simulink model "sm_car"  (R2025a)
settings: Solver=ode23t  StartTime=0.0  StopTime=400  MaxStep=0.4  RelTol=1e-3  AbsTol=1e-3  EnableMultiTasking=on
PreLoadFcn:
  | % Due to usability issue in Repeating Sequence block
  | warning('off','Simulink:Masking:Invalid');
  | 
  | % Eliminate unnecessary warnings in inactive variants
  | % Warnings generated only if you click through inactive variant
  | warning('off','MATLAB:nonExistentField');
  | warning('off','Simulink:Parameters:BlkParamUndefined');
PostLoadFcn:
  | set_param([bdroot '/Vehicle'],'popup_trailer','Off')
  | warning('off','sm:sli:setup:compile:LocalSolverNotSupported')
  | %sm_car_config_maneuver(bdroot,'WOT Braking');
  | sm_car_config_vehicle(bdroot,'false');
  | sm_car_config_logging(bdroot);
InitFcn:
  | sm_car_config_camera;
  | Vehicle = sm_car_vehcfg_checkConfig(Vehicle);
  | sm_car_check_tire_model(bdroot);
StartFcn:
  | tic;
StopFcn:
  | Elapsed_Sim_Time = toc;
  | % disp(['Elapsed Sim Time = ' num2str(Elapsed_Sim_Time)]);
undefined symbols (not defined in the file): Axle1D, AxleIn, Camera, Control, Driver, Free, Init, Maneuver, Pedal, RaceFix, RaceSpin, Scene, ShaftL1, ShaftL2, ShaftR1, ShaftR2, Soft, Stiff, Visual, X, xy_data_car_side, Y, Z
libraries: sm_lib x1546, nesl_utility x528, fl_lib x480, SimscapeFluids_lib x61, sdl_lib x49, simulink x29, ee_lib x7, simulink_extras x6, Linkage_Systems x4, Tire_1x2x x4, AntiRollBar_Systems x2, Linkage_Decoupled x2
(part 2 of 79)

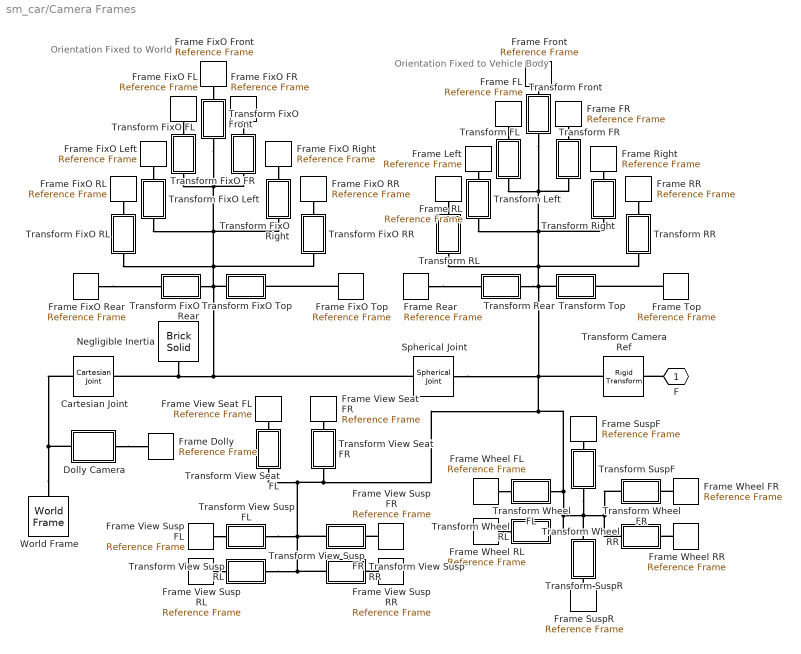
== system sm_car/Camera Frames ==
  note: Orientation Fixed to World
  note: Orientation Fixed to Vehicle Body
  Cartesian Joint : sm_lib/Joints/Cartesian Joint  JointMode=Normal  CompositeWrenchDir=FollowerOnBase  CompositeWrenchFrame=BaseFrame  SenseConstraintForce=off  SenseConstraintTorque=off  SenseTotalForce=off  SenseTotalTorque=off  PxPositionTargetSpecify=off  PxPositionTargetPriority=High  PxPositionTargetValue=0  PxPositionTargetValueUnits=m  PxVelocityTargetSpecify=off  PxVelocityTargetPriority=High  PxVelocityTargetValue=0  PxVelocityTargetValueUnits=m/s  PxEquilibriumPosition=0  PxEquilibriumPositionUnits=m  PxSpringStiffness=0  PxSpringStiffnessUnits=N/m  PxDampingCoefficient=0  PxDampingCoefficientUnits=N/(m/s)  PxLowerLimitSpecify=off  PxLowerLimitBound=-1  PxLowerLimitBoundUnits=m  PxLowerLimitStiffness=1e6  PxLowerLimitStiffnessUnits=N/m  PxLowerLimitDamping=1e3  PxLowerLimitDampingUnits=N/(m/s)  PxLowerLimitTransitionRegionWidth=1e-4  PxLowerLimitTransitionRegionWidthUnits=m  PxUpperLimitSpecify=off  PxUpperLimitBound=1  PxUpperLimitBoundUnits=m  PxUpperLimitStiffness=1e6  PxUpperLimitStiffnessUnits=N/m  PxUpperLimitDamping=1e3  PxUpperLimitDampingUnits=N/(m/s)  PxUpperLimitTransitionRegionWidth=1e-4  PxUpperLimitTransitionRegionWidthUnits=m  PxTorqueActuationMode=NoTorque  PxMotionActuationMode=ComputedMotion  PxSensePosition=off  PxSenseVelocity=off  PxSenseAcceleration=off  PxSenseTorqueForce=off  PxSenseLowerLimitTorqueForce=off  PxSenseUpperLimitTorqueForce=off  PyPositionTargetSpecify=off  PyPositionTargetPriority=High  PyPositionTargetValue=0  PyPositionTargetValueUnits=m  PyVelocityTargetSpecify=off  PyVelocityTargetPriority=High  PyVelocityTargetValue=0  PyVelocityTargetValueUnits=m/s  PyEquilibriumPosition=0  PyEquilibriumPositionUnits=m  PySpringStiffness=0  PySpringStiffnessUnits=N/m  PyDampingCoefficient=0  PyDampingCoefficientUnits=N/(m/s)  PyLowerLimitSpecify=off  PyLowerLimitBound=-1  PyLowerLimitBoundUnits=m  PyLowerLimitStiffness=1e6  PyLowerLimitStiffnessUnits=N/m  PyLowerLimitDamping=1e3  PyLowerLimitDampingUnits=N/(m/s)  PyLowerLimitTransitionRegionWidth=1e-4  PyLowerLimitTransitionRegionWidthUnits=m  PyUpperLimitSpecify=off  PyUpperLimitBound=1  PyUpperLimitBoundUnits=m  PyUpperLimitStiffness=1e6  PyUpperLimitStiffnessUnits=N/m  PyUpperLimitDamping=1e3  PyUpperLimitDampingUnits=N/(m/s)  PyUpperLimitTransitionRegionWidth=1e-4  PyUpperLimitTransitionRegionWidthUnits=m  PyTorqueActuationMode=NoTorque  PyMotionActuationMode=ComputedMotion  PySensePosition=off  PySenseVelocity=off  PySenseAcceleration=off  PySenseTorqueForce=off  PySenseLowerLimitTorqueForce=off  PySenseUpperLimitTorqueForce=off  PzPositionTargetSpecify=off  PzPositionTargetPriority=High  PzPositionTargetValue=0  PzPositionTargetValueUnits=m  PzVelocityTargetSpecify=off  PzVelocityTargetPriority=High  PzVelocityTargetValue=0  PzVelocityTargetValueUnits=m/s  PzEquilibriumPosition=0  PzEquilibriumPositionUnits=m  PzSpringStiffness=0  PzSpringStiffnessUnits=N/m  PzDampingCoefficient=0  PzDampingCoefficientUnits=N/(m/s)  PzLowerLimitSpecify=off  PzLowerLimitBound=-1  PzLowerLimitBoundUnits=m  PzLowerLimitStiffness=1e6  PzLowerLimitStiffnessUnits=N/m  PzLowerLimitDamping=1e3  PzLowerLimitDampingUnits=N/(m/s)  PzLowerLimitTransitionRegionWidth=1e-4  PzLowerLimitTransitionRegionWidthUnits=m  PzUpperLimitSpecify=off  PzUpperLimitBound=1  PzUpperLimitBoundUnits=m  PzUpperLimitStiffness=1e6  PzUpperLimitStiffnessUnits=N/m  PzUpperLimitDamping=1e3  PzUpperLimitDampingUnits=N/(m/s)  PzUpperLimitTransitionRegionWidth=1e-4  PzUpperLimitTransitionRegionWidthUnits=m  PzTorqueActuationMode=NoTorque  PzMotionActuationMode=ComputedMotion  PzSensePosition=off  PzSenseVelocity=off  PzSenseAcceleration=off  PzSenseTorqueForce=off  PzSenseLowerLimitTorqueForce=off  PzSenseUpperLimitTorqueForce=off
  Dolly Camera : Subsystem  Variant=on  VariantControlMode=label  VariantControl=Variant1  LabelModeActiveChoice=Off
      settings: AttributesFormatString=%<ActiveVariant>
      mask Display: disp(' ');
  Frame Dolly : sm_lib/Frames and Transforms/Reference Frame
  Frame FL : sm_lib/Frames and Transforms/Reference Frame
  Frame FR : sm_lib/Frames and Transforms/Reference Frame
  Frame FixO FL : sm_lib/Frames and Transforms/Reference Frame
  Frame FixO FR : sm_lib/Frames and Transforms/Reference Frame
  Frame FixO Front : sm_lib/Frames and Transforms/Reference Frame
  Frame FixO Left : sm_lib/Frames and Transforms/Reference Frame
  Frame FixO RL : sm_lib/Frames and Transforms/Reference Frame
  Frame FixO RR : sm_lib/Frames and Transforms/Reference Frame
  Frame FixO Rear : sm_lib/Frames and Transforms/Reference Frame
  Frame FixO Right : sm_lib/Frames and Transforms/Reference Frame
  Frame FixO Top : sm_lib/Frames and Transforms/Reference Frame
  Frame Front : sm_lib/Frames and Transforms/Reference Frame
  Frame Left : sm_lib/Frames and Transforms/Reference Frame
  Frame RL : sm_lib/Frames and Transforms/Reference Frame
  Frame RR : sm_lib/Frames and Transforms/Reference Frame
  Frame Rear : sm_lib/Frames and Transforms/Reference Frame
  Frame Right : sm_lib/Frames and Transforms/Reference Frame
  Frame SuspF : sm_lib/Frames and Transforms/Reference Frame
  Frame SuspR : sm_lib/Frames and Transforms/Reference Frame
  Frame Top : sm_lib/Frames and Transforms/Reference Frame
  Frame View Seat FL : sm_lib/Frames and Transforms/Reference Frame
  Frame View Seat FR : sm_lib/Frames and Transforms/Reference Frame
  Frame View Susp FL : sm_lib/Frames and Transforms/Reference Frame
  Frame View Susp FR : sm_lib/Frames and Transforms/Reference Frame
  Frame View Susp RL : sm_lib/Frames and Transforms/Reference Frame
  Frame View Susp RR : sm_lib/Frames and Transforms/Reference Frame
  Frame Wheel FL : sm_lib/Frames and Transforms/Reference Frame
  Frame Wheel FR : sm_lib/Frames and Transforms/Reference Frame
  Frame Wheel RL : sm_lib/Frames and Transforms/Reference Frame
  Frame Wheel RR : sm_lib/Frames and Transforms/Reference Frame
  Negligible Inertia : sm_lib/Body Elements/Brick Solid  BrickDimensions=[1 1 1]*1e-3  BrickDimensionsUnits=m  ExportEntireGeometry=off  InertiaType=PointMass  BasedOnType=Density  Density=1000  DensityUnits=kg/m^3  Mass=1e-6  MassUnits=kg  CenterOfMass=[0 0 0]  CenterOfMassUnits=m  MomentsOfInertia=[1 1 1]  MomentsOfInertiaUnits=kg*m^2  ProductsOfInertia=[1 1 1]  ProductsOfInertiaUnits=kg*m^2  GraphicType=FromGeometry  MarkerShape=Sphere  MarkerSize=10  GraphicVisPropType=SimpleVisualProperties  GraphicDiffuseColor=[0.5 0.5 0.5]  GraphicOpacity=1.0  GraphicSpecularColor=[0.5 0.5 0.5 1.0]  GraphicAmbientColor=[0.15 0.15 0.15 1.0]  GraphicEmissiveColor=[0.0 0.0 0.0 1.0]  GraphicShininess=75  DoExposeReferenceFrame=on  SerializedFrames=<Frames/>
  Spherical Joint : sm_lib/Joints/Spherical Joint  JointMode=Normal  CompositeWrenchDir=FollowerOnBase  CompositeWrenchFrame=BaseFrame  SenseConstraintForce=off  SenseConstraintTorque=off  SenseTotalForce=off  SenseTotalTorque=off  PositionTargetSpecify=off  PositionTargetPriority=High  PositionTargetRotationMethod=None  PositionTargetFollAlignAxisA=+X  PositionTargetBaseAlignAxisA=+Y  PositionTargetFollAlignAxisB=+Y  PositionTargetBaseAlignAxisB=+Z  PositionTargetRotationStandardAxis=+Z  PositionTargetRotationAngle=0.0  PositionTargetRotationAngleUnits=deg  PositionTargetRotationArbitraryAxis=[0 0 1]  PositionTargetRotationSequenceAxes=FollowerAxes  PositionTargetRotationSequence=XYX  PositionTargetRotationSequenceAngles=[0 0 0]  PositionTargetRotationSequenceAnglesUnits=deg  PositionTargetRotationMatrix=[1 0 0; 0 1 0; 0 0 1]  PositionTargetQuaternion=[1 0 0 0]  VelocityTargetSpecify=off  VelocityTargetPriority=High  VelocityTargetValue=[0 0 0]  VelocityTargetValueUnits=deg/s  VelocityTargetInFollowerFrame=on  EqPosRotationMethod=None  EqPosFollAlignAxisA=+X  EqPosBaseAlignAxisA=+Y  EqPosFollAlignAxisB=+Y  EqPosBaseAlignAxisB=+Z  EqPosRotationStandardAxis=+Z  EqPosRotationAngle=0.0  EqPosRotationAngleUnits=deg  EqPosRotationArbitraryAxis=[0 0 1]  EqPosRotationSequenceAxes=FollowerAxes  EqPosRotationSequence=XYX  EqPosRotationSequenceAngles=[0 0 0]  EqPosRotationSequenceAnglesUnits=deg  EqPosRotationMatrix=[1 0 0; 0 1 0; 0 0 1]  EqPosQuaternion=[1 0 0 0]  SpringStiffness=0  SpringStiffnessUnits=N*m/deg  DampingCoefficient=0  DampingCoefficientUnits=N*m/(deg/s)  LowerLimitSpecify=off  LowerLimitBound=15  LowerLimitBoundUnits=deg  LowerLimitStiffness=1e4  LowerLimitStiffnessUnits=N*m/deg  LowerLimitDamping=10  LowerLimitDampingUnits=N*m/(deg/s)  LowerLimitTransitionRegionWidth=0.1  LowerLimitTransitionRegionWidthUnits=deg  UpperLimitSpecify=off  UpperLimitBound=45  UpperLimitBoundUnits=deg  UpperLimitStiffness=1e4  UpperLimitStiffnessUnits=N*m/deg  UpperLimitDamping=10  UpperLimitDampingUnits=N*m/(deg/s)  UpperLimitTransitionRegionWidth=0.1  UpperLimitTransitionRegionWidthUnits=deg  TorqueActuationMode=NoTorque  ActuateTorqueX=off  ActuateTorqueY=off  ActuateTorqueZ=off  ActuateTorque=off  ActuationFrame=BaseFrame  SensePosition=off  SenseVelocityX=off  SenseVelocityY=off  SenseVelocityZ=off  SenseVelocity=off  SenseAccelerationX=off  SenseAccelerationY=off  SenseAccelerationZ=off  SenseAcceleration=off  SenseLowerLimitTorqueMag=off  SenseUpperLimitTorqueMag=off  SensingFrame=BaseFrame
  Transform Camera Ref : sm_lib/Frames and Transforms/Rigid Transform  RotationMethod=RotationSequence  FollAlignAxisA=+X  BaseAlignAxisA=+Y  FollAlignAxisB=+Y  BaseAlignAxisB=+Z  RotationStandardAxis=+Z  RotationAngle=0.0  RotationAngleUnits=deg  RotationArbitraryAxis=[0 0 1]  RotationSequenceAxes=FollowerAxes  RotationSequence=ZYX  RotationSequenceAngles=[Camera.Offset.a.Value(3) Camera.Offset.a.Value(2) Camera.Offset.a.Value(1)]  RotationSequenceAnglesUnits=deg  RotationMatrix=[1 0 0; 0 1 0; 0 0 1]  Quaternion=[1 0 0 0]  TranslationMethod=Cartesian  TranslationCartesianOffset=Camera.Offset.s.Value  TranslationCartesianOffsetUnits=m  TranslationStandardAxis=+Z  TranslationStandardOffset=0  TranslationStandardOffsetUnits=m  TranslationROffset=0  TranslationROffsetUnits=m  TranslationThetaOffset=0  TranslationThetaOffsetUnits=deg  TranslationZOffset=0  TranslationZOffsetUnits=m
  Transform FL : Subsystem  mask(Define Camera Frame){CF=Camera.FL}
      mask prompts: CF "Camera Frame Data (structure)"
      mask help: Sets frame position and orientation for camera frame. Data structure provides cartesian location and orientation. Orientation is intrinsic rotation of yaw-pitch-roll.
  Transform FR : Subsystem  mask(Define Camera Frame){CF=Camera.FR}
      mask prompts: CF "Camera Frame Data (structure)"
      mask help: Sets frame position and orientation for camera frame. Data structure provides cartesian location and orientation. Orientation is intrinsic rotation of yaw-pitch-roll.
  Transform FixO FL : Subsystem  mask(Define Camera Frame){CF=Camera.FL}
      mask prompts: CF "Camera Frame Data (structure)"
      mask help: Sets frame position and orientation for camera frame. Data structure provides cartesian location and orientation. Orientation is intrinsic rotation of yaw-pitch-roll.
  Transform FixO FR : Subsystem  mask(Define Camera Frame){CF=Camera.FR}
      mask prompts: CF "Camera Frame Data (structure)"
      mask help: Sets frame position and orientation for camera frame. Data structure provides cartesian location and orientation. Orientation is intrinsic rotation of yaw-pitch-roll.
  Transform FixO Front : Subsystem  mask(Define Camera Frame){CF=Camera.Front}
      mask prompts: CF "Camera Frame Data (structure)"
      mask help: Sets frame position and orientation for camera frame. Data structure provides cartesian location and orientation. Orientation is intrinsic rotation of yaw-pitch-roll.
  Transform FixO Left : Subsystem  mask(Define Camera Frame){CF=Camera.Left}
      mask prompts: CF "Camera Frame Data (structure)"
      mask help: Sets frame position and orientation for camera frame. Data structure provides cartesian location and orientation. Orientation is intrinsic rotation of yaw-pitch-roll.
  Transform FixO RL : Subsystem  mask(Define Camera Frame){CF=Camera.RL}
      mask prompts: CF "Camera Frame Data (structure)"
      mask help: Sets frame position and orientation for camera frame. Data structure provides cartesian location and orientation. Orientation is intrinsic rotation of yaw-pitch-roll.
  Transform FixO RR : Subsystem  mask(Define Camera Frame){CF=Camera.RR}
      mask prompts: CF "Camera Frame Data (structure)"
      mask help: Sets frame position and orientation for camera frame. Data structure provides cartesian location and orientation. Orientation is intrinsic rotation of yaw-pitch-roll.
  Transform FixO Rear : Subsystem  mask(Define Camera Frame){CF=Camera.Rear}
      mask prompts: CF "Camera Frame Data (structure)"
      mask help: Sets frame position and orientation for camera frame. Data structure provides cartesian location and orientation. Orientation is intrinsic rotation of yaw-pitch-roll.
  Transform FixO Right : Subsystem  mask(Define Camera Frame){CF=Camera.Right}
      mask prompts: CF "Camera Frame Data (structure)"
      mask help: Sets frame position and orientation for camera frame. Data structure provides cartesian location and orientation. Orientation is intrinsic rotation of yaw-pitch-roll.
  Transform FixO Top : Subsystem  mask(Define Camera Frame){CF=Camera.Top}
      mask prompts: CF "Camera Frame Data (structure)"
      mask help: Sets frame position and orientation for camera frame. Data structure provides cartesian location and orientation. Orientation is intrinsic rotation of yaw-pitch-roll.
  Transform Front : Subsystem  mask(Define Camera Frame){CF=Camera.Front}
      mask prompts: CF "Camera Frame Data (structure)"
      mask help: Sets frame position and orientation for camera frame. Data structure provides cartesian location and orientation. Orientation is intrinsic rotation of yaw-pitch-roll.
  Transform Left : Subsystem  mask(Define Camera Frame){CF=Camera.Left}
      mask prompts: CF "Camera Frame Data (structure)"
      mask help: Sets frame position and orientation for camera frame. Data structure provides cartesian location and orientation. Orientation is intrinsic rotation of yaw-pitch-roll.
  Transform RL : Subsystem  mask(Define Camera Frame){CF=Camera.RL}
      mask prompts: CF "Camera Frame Data (structure)"
      mask help: Sets frame position and orientation for camera frame. Data structure provides cartesian location and orientation. Orientation is intrinsic rotation of yaw-pitch-roll.
  Transform RR : Subsystem  mask(Define Camera Frame){CF=Camera.RR}
      mask prompts: CF "Camera Frame Data (structure)"
      mask help: Sets frame position and orientation for camera frame. Data structure provides cartesian location and orientation. Orientation is intrinsic rotation of yaw-pitch-roll.
  Transform Rear : Subsystem  mask(Define Camera Frame){CF=Camera.Rear}
      mask prompts: CF "Camera Frame Data (structure)"
      mask help: Sets frame position and orientation for camera frame. Data structure provides cartesian location and orientation. Orientation is intrinsic rotation of yaw-pitch-roll.
  Transform Right : Subsystem  mask(Define Camera Frame){CF=Camera.Right}
      mask prompts: CF "Camera Frame Data (structure)"
      mask help: Sets frame position and orientation for camera frame. Data structure provides cartesian location and orientation. Orientation is intrinsic rotation of yaw-pitch-roll.
  Transform SuspF : Subsystem  mask(Define Camera Frame){CF=Camera.SuspF}
      mask prompts: CF "Camera Frame Data (structure)"
      mask help: Sets frame position and orientation for camera frame. Data structure provides cartesian location and orientation. Orientation is intrinsic rotation of yaw-pitch-roll.
  Transform SuspR : Subsystem  mask(Define Camera Frame){CF=Camera.SuspR}
      mask prompts: CF "Camera Frame Data (structure)"
      mask help: Sets frame position and orientation for camera frame. Data structure provides cartesian location and orientation. Orientation is intrinsic rotation of yaw-pitch-roll.
  Transform Top : Subsystem  mask(Define Camera Frame){CF=Camera.Top}
      mask prompts: CF "Camera Frame Data (structure)"
      mask help: Sets frame position and orientation for camera frame. Data structure provides cartesian location and orientation. Orientation is intrinsic rotation of yaw-pitch-roll.
  Transform View Seat FL : Subsystem  mask(Define Camera Frame){CF=Camera.View_SeatFL}
      mask prompts: CF "Camera Frame Data (structure)"
      mask help: Sets frame position and orientation for camera frame. Data structure provides cartesian location and orientation. Orientation is intrinsic rotation of yaw-pitch-roll.
  Transform View Seat FR : Subsystem  mask(Define Camera Frame){CF=Camera.View_SeatFR}
      mask prompts: CF "Camera Frame Data (structure)"
      mask help: Sets frame position and orientation for camera frame. Data structure provides cartesian location and orientation. Orientation is intrinsic rotation of yaw-pitch-roll.
  Transform View Susp FL : Subsystem  mask(Define Camera Frame){CF=Camera.View_SuspFL}
      mask prompts: CF "Camera Frame Data (structure)"
      mask help: Sets frame position and orientation for camera frame. Data structure provides cartesian location and orientation. Orientation is intrinsic rotation of yaw-pitch-roll.
  Transform View Susp FR : Subsystem  mask(Define Camera Frame){CF=Camera.View_SuspFR}
      mask prompts: CF "Camera Frame Data (structure)"
      mask help: Sets frame position and orientation for camera frame. Data structure provides cartesian location and orientation. Orientation is intrinsic rotation of yaw-pitch-roll.
  Transform View Susp RL : Subsystem  mask(Define Camera Frame){CF=Camera.View_SuspRL}
      mask prompts: CF "Camera Frame Data (structure)"
      mask help: Sets frame position and orientation for camera frame. Data structure provides cartesian location and orientation. Orientation is intrinsic rotation of yaw-pitch-roll.
  Transform View Susp RR : Subsystem  mask(Define Camera Frame){CF=Camera.View_SuspRR}
      mask prompts: CF "Camera Frame Data (structure)"
      mask help: Sets frame position and orientation for camera frame. Data structure provides cartesian location and orientation. Orientation is intrinsic rotation of yaw-pitch-roll.
  Transform Wheel FL : Subsystem  mask(Define Camera Frame){CF=Camera.Wheel_FL}
      mask prompts: CF "Camera Frame Data (structure)"
      mask help: Sets frame position and orientation for camera frame. Data structure provides cartesian location and orientation. Orientation is intrinsic rotation of yaw-pitch-roll.
  Transform Wheel FR : Subsystem  mask(Define Camera Frame){CF=Camera.Wheel_FR}
      mask prompts: CF "Camera Frame Data (structure)"
      mask help: Sets frame position and orientation for camera frame. Data structure provides cartesian location and orientation. Orientation is intrinsic rotation of yaw-pitch-roll.
  Transform Wheel RL : Subsystem  mask(Define Camera Frame){CF=Camera.Wheel_RL}
      mask prompts: CF "Camera Frame Data (structure)"
      mask help: Sets frame position and orientation for camera frame. Data structure provides cartesian location and orientation. Orientation is intrinsic rotation of yaw-pitch-roll.
  Transform Wheel RR : Subsystem  mask(Define Camera Frame){CF=Camera.Wheel_RR}
      mask prompts: CF "Camera Frame Data (structure)"
      mask help: Sets frame position and orientation for camera frame. Data structure provides cartesian location and orientation. Orientation is intrinsic rotation of yaw-pitch-roll.
  World Frame : sm_lib/Frames and Transforms/World Frame
  F : PMIOPort  Side=Right
  connections:
  Dolly Camera/RConn1 -- Frame Dolly/RConn1
  Frame View Susp RL/RConn1 -- Transform View Susp RL/RConn1
  Frame View Susp RR/RConn1 -- Transform View Susp RR/RConn1
  Frame View Susp FR/RConn1 -- Transform View Susp FR/RConn1
  Frame View Susp FL/RConn1 -- Transform View Susp FL/RConn1
  Frame View Seat FR/RConn1 -- Transform View Seat FR/RConn1
  Frame View Seat FL/RConn1 -- Transform View Seat FL/RConn1
  Frame Wheel RL/RConn1 -- Transform Wheel RL/RConn1
  Frame Wheel FL/RConn1 -- Transform Wheel FL/RConn1
  Frame Wheel RR/RConn1 -- Transform Wheel RR/RConn1
  Frame Wheel FR/RConn1 -- Transform Wheel FR/RConn1
  Frame SuspR/RConn1 -- Transform SuspR/RConn1
  Frame SuspF/RConn1 -- Transform SuspF/RConn1
  Frame Front/RConn1 -- Transform Front/RConn1
  Frame RR/RConn1 -- Transform RR/RConn1
  Frame FR/RConn1 -- Transform FR/RConn1
  Frame Right/RConn1 -- Transform Right/RConn1
  Frame RL/RConn1 -- Transform RL/RConn1
  Frame FL/RConn1 -- Transform FL/RConn1
  Frame Left/RConn1 -- Transform Left/RConn1
  Frame Top/RConn1 -- Transform Top/RConn1
  Frame Rear/RConn1 -- Transform Rear/RConn1
  Frame FixO Rear/RConn1 -- Transform FixO Rear/RConn1
  Frame FixO Front/RConn1 -- Transform FixO Front/RConn1
  Frame FixO Top/RConn1 -- Transform FixO Top/RConn1
  Frame FixO FL/RConn1 -- Transform FixO FL/RConn1
  Frame FixO Left/RConn1 -- Transform FixO Left/RConn1
  Frame FixO RL/RConn1 -- Transform FixO RL/RConn1
  Frame FixO RR/RConn1 -- Transform FixO RR/RConn1
  Frame FixO Right/RConn1 -- Transform FixO Right/RConn1
  Frame FixO FR/RConn1 -- Transform FixO FR/RConn1
  Transform FixO RL/LConn1 -- Transform FixO RR/LConn1 -- Transform FixO Left/LConn1 -- Transform FixO Right/LConn1 -- Transform FixO FR/LConn1 -- Transform FixO Front/LConn1 -- Transform FixO FL/LConn1 -- Transform FixO Top/LConn1 -- Transform FixO Rear/LConn1 -- Spherical Joint/LConn1 -- Cartesian Joint/RConn1 -- Negligible Inertia/RConn1
  World Frame/RConn1 -- Cartesian Joint/LConn1 -- Dolly Camera/LConn1
  Transform View Susp FL/LConn1 -- Transform View Seat FL/LConn1 -- Transform Rear/LConn1 -- Transform FL/LConn1 -- Transform Front/LConn1 -- Transform FR/LConn1 -- Transform Right/LConn1 -- Transform Left/LConn1 -- Transform RR/LConn1 -- Transform RL/LConn1 -- Transform Top/LConn1 -- Transform Camera Ref/RConn1 -- Spherical Joint/RConn1 -- Transform Wheel FL/LConn1 -- Transform Wheel RL/LConn1 -- Transform SuspF/LConn1 -- Transform SuspR/LConn1 -- Transform Wheel FR/LConn1 -- Transform Wheel RR/LConn1 -- Transform View Seat FR/LConn1 -- Transform View Susp RR/LConn1 -- Transform View Susp RL/LConn1 -- Transform View Susp FR/LConn1
  F/RConn1 -- Transform Camera Ref/LConn1

== system sm_car/Check ==
  l : Inport
  v : Inport  Port=2
  Bus Selector : BusSelector  OutputSignals=World.vx,World.vy  OutputAsBus=on
  Bus Selector1 : BusSelector  OutputSignals=Reference.latdev,Reference.nLap,Reference.dist
  End Distance : Constant  Value=max_dist_threshold
  End Lap : Constant  Value=end_lap_num
  Lateral Deviation Threshold : Constant  Value=lat_dev_threshold
  Less Than : RelationalOperator  Operator=<  OutDataTypeStr=boolean  RndMeth=Simplest  InputSameDT=off
  Less Than1 : RelationalOperator  Operator=>  OutDataTypeStr=boolean  ZeroCross=off  RndMeth=Simplest  InputSameDT=off
  Less Than2 : RelationalOperator  OutDataTypeStr=boolean  RndMeth=Simplest  InputSameDT=off
  Less Than3 : RelationalOperator  Operator=>  OutDataTypeStr=boolean  RndMeth=Simplest  InputSameDT=off
  Less Than4 : RelationalOperator  Operator=>  OutDataTypeStr=boolean  ZeroCross=off  RndMeth=Simplest  InputSameDT=off
  Max Speed Threshold : Constant  Value=max_speed
  Product{,1..4} (5 alike) : Product
  Start Checking : Step  Time=start_check_time  SampleTime=0  ZeroCross=off
  Start Checking End Distance : Step  Time=start_check_time_max_dist  SampleTime=0  ZeroCross=off
  Start Checking End Lap : Step  Time=start_check_time_end_lap  SampleTime=0  ZeroCross=off
  Start Checking Lat Dev : Step  Time=start_check_time_ld  SampleTime=0  ZeroCross=off
  Start Checking Max Speed : Step  Time=start_check_time_max_speed  SampleTime=0  ZeroCross=off
  Stop Threshold : Constant  Value=stop_speed
  Sum : Sum  Inputs=+++++
  Vel in xy plane : Fcn  Expr=sqrt(u(1)^2+u(2)^2)
  Stop : Outport  VectorParamsAs1DForOutWhenUnconnected=off
  wires:
  Product4/1 -> Sum/5
  Start Checking End Distance/1 -> Product4/2
  Less Than4/1 -> Product4/1
  Bus Selector1/3 -> Less Than4/1  "<dist>"
  End Distance/1 -> Less Than4/2
  Less Than/1 -> Product/1
  Stop Threshold/1 -> Less Than/2
  v/1 -> Bus Selector/1
  Start Checking/1 -> Product/2
  Product/1 -> Sum/1
  Bus Selector/1 -> Vel in xy plane/1
  Vel in xy plane/1 -> Less Than/1, Less Than3/1  "speed"
  l/1 -> Bus Selector1/1
  Bus Selector1/1 -> Less Than1/1  "<latdev>"
  Lateral Deviation Threshold/1 -> Less Than1/2
  Less Than1/1 -> Product1/1
  Start Checking Lat Dev/1 -> Product1/2
  Sum/1 -> Stop/1
  Product1/1 -> Sum/3
  End Lap/1 -> Less Than2/2
  Less Than2/1 -> Product2/1
  Start Checking End Lap/1 -> Product2/2
  Product2/1 -> Sum/4
  Start Checking Max Speed/1 -> Product3/2
  Less Than3/1 -> Product3/1
  Max Speed Threshold/1 -> Less Than3/2
  Product3/1 -> Sum/2
  Bus Selector1/2 -> Less Than2/1  "<nLap>"

== system sm_car/Controller ==
  "DrvBus " : Inport
  "VehBus " : Inport  Port=2
  Default : Subsystem  VariantControl=Default  mask{popup_brake_control=Pedal, popup_damper_control_A1=None, popup_damper_control_A2=None, popup_spring_control_A1=None, popup_gas_spring_A1=Soft, popup_spring_control_A2=None, popup_gas_spring_A2=Soft}
      mask prompts: popup_brake_control "Control Type"; popup_damper_control_A1 "Damper Control Axle 1"; popup_damper_control_A2 "Damper Control Axle 2"; popup_spring_control_A1 "Spring Control Axle 1"; popup_gas_spring_A1 "Gas Spring (Axle 1)"; popup_spring_control_A2 "Spring Control Axle 2"; popup_gas_spring_A2 "Gas Spring (Axle 2)"
      mask TypeOptions popup_brake_control: Brake Control/popup_brake_control
      mask TypeOptions popup_damper_control_A1: Damper Control/popup_damper_control_A1
      mask TypeOptions popup_damper_control_A2: Damper Control/popup_damper_control_A2
      mask TypeOptions popup_spring_control_A1: Spring Control/popup_spring_control_A1
      mask Callback popup_spring_control_A1:
      | bh = gcb;
      | maskObj = Simulink.Mask.get(bh); % Get the mask object of the current block
      | psg_h   = maskObj.getParameter('popup_gas_spring_A1'); % Get the parameter to hide
      | 
      | % Check the value of ControlParam
      | controlParamValue = get_param(bh, 'popup_spring_control_A1');
      | 
      | psg_h.Visible  = 'off';
      | 
      | if strcmp(controlParamValue, 'Hydropneumatic')
      |     psg_h.Visible  = 'on';
      | else
      |     psg_h.Visible  = 'off';
      | end
      mask TypeOptions popup_gas_spring_A1: Spring Control/popup_gas_spring_A1
      mask TypeOptions popup_spring_control_A2: Spring Control/popup_spring_control_A2
      mask Callback popup_spring_control_A2:
      | bh = gcb;
      | maskObj = Simulink.Mask.get(bh); % Get the mask object of the current block
      | psg_h   = maskObj.getParameter('popup_gas_spring_A2'); % Get the parameter to hide
      | 
      | % Check the value of ControlParam
      | controlParamValue = get_param(bh, 'popup_spring_control_A2');
      | 
      | psg_h.Visible  = 'off';
      | 
      | if strcmp(controlParamValue, 'Hydropneumatic')
      |     psg_h.Visible  = 'on';
      | else
      |     psg_h.Visible  = 'off';
      | end
      mask TypeOptions popup_gas_spring_A2: Spring Control/popup_gas_spring_A2
  TrqVec 4Motor : Subsystem  VariantControl=TrqVec_4Motor  mask{popup_brake_control=Pedal, popup_damper_control_A1=None, popup_damper_control_A2=None, popup_spring_control_A1=None, popup_spring_control_A2=None}
      mask prompts: popup_brake_control "Control Type"; popup_damper_control_A1 "Damper Control Axle 1"; popup_damper_control_A2 "Damper Control Axle 2"; popup_spring_control_A1 "Spring Control Axle 1"; popup_spring_control_A2 "Spring Control Axle 2"
      mask TypeOptions popup_brake_control: Brake Control/popup_brake_control
      mask TypeOptions popup_damper_control_A1: Damper Control/popup_damper_control_A1
      mask TypeOptions popup_damper_control_A2: Damper Control/popup_damper_control_A2
      mask TypeOptions popup_spring_control_A1: Spring Control/popup_spring_control_A1
      mask TypeOptions popup_spring_control_A2: Spring Control/popup_spring_control_A2
  " CtrlBus" : Outport  VectorParamsAs1DForOutWhenUnconnected=off

== system sm_car/Driver ==
  "VehBus " : Inport
  Obs : Inport  Port=2
  Closed Loop : Subsystem  VariantControl=Closed_Loop
  Open Loop : Subsystem  VariantControl=Open_Loop
  " DrvBus" : Outport  VectorParamsAs1DForOutWhenUnconnected=off

== system sm_car/Road ==
  VehBus : Inport
  Bus Creator : BusCreator  Inputs=6
  Bus Selector1 : BusSelector  OutputSignals=Chassis
  Ground : Subsystem
  Input fWindCar : Subsystem  mask{fWind=[0 0 0], tWind=2, dWind=30000}
      mask prompts: fWind "Force [x y z] (N)"; tWind "Duration (s)"; dWind "Start time (sec)"
  Input fWindTrailer : Subsystem  mask{fWind=[0 0 0], tWind=2, dWind=30000}
      mask prompts: fWind "Force [x y z] (N)"; tWind "Duration (s)"; dWind "Start time (sec)"
  Mu Scaling by Position : Subsystem  mask(Scale Friction Coefficient by Position){muFL_out=1, muFR_out=1, muRL_out=1, muRR_out=1, muFL_in=1, muFR_in=1, muRL_in=1, muRR_in=1, intvX_FL_start=100-40, intvX_FR_start=100-40, intvX_RL_start=100-40, intvX_RR_start=100-40, intvX_FL_end=130-40, intvX_FR_end=130-40, intvX_RL_end=130-40, intvX_RR_end=130-40, intvY_FL_start=-30, intvY_FR_start=-30, intvY_RL_start=-30, intvY_RR_start=-30, intvY_FL_end=0, intvY_FR_end=0, intvY_RL_end=0, intvY_RR_end=0}
      mask help: Models a rectangular patch with a unique coefficient of friction. If the wheel xy-position is inside the rectangular patch, a different scaling factor is applied to the road coefficients of friction along x and y.
      mask TypeOptions muFL_out: muFL out/Value
      mask TypeOptions muFR_out: muFR out/Value
      mask TypeOptions muRL_out: muRL out/Value
      mask TypeOptions muRR_out: muRR out/Value
      mask TypeOptions muFL_in: muFL in/Value
      mask TypeOptions muFR_in: muFR in/Value
      mask TypeOptions muRL_in: muRL in/Value
      mask TypeOptions muRR_in: muRR in/Value
      mask TypeOptions intvX_FL_start: Interval Test FLx/lowlimit
      mask TypeOptions intvX_FR_start: Interval Test FRx/lowlimit
      mask TypeOptions intvX_RL_start: Interval Test RLx/lowlimit
      mask TypeOptions intvX_RR_start: Interval Test RRx/lowlimit
      mask TypeOptions intvX_FL_end: Interval Test FLx/uplimit
      mask TypeOptions intvX_FR_end: Interval Test FRx/uplimit
      mask TypeOptions intvX_RL_end: Interval Test RLx/uplimit
      mask TypeOptions intvX_RR_end: Interval Test RRx/uplimit
      mask TypeOptions intvY_FL_start: Interval Test FLy/lowlimit
      mask TypeOptions intvY_FR_start: Interval Test FRy/lowlimit
      mask TypeOptions intvY_RL_start: Interval Test RLy/lowlimit
      mask TypeOptions intvY_RR_start: Interval Test RRy/lowlimit
      mask TypeOptions intvY_FL_end: Interval Test FLy/uplimit
      mask TypeOptions intvY_FR_end: Interval Test FRy/uplimit
      mask TypeOptions intvY_RL_end: Interval Test RLy/uplimit
      mask TypeOptions intvY_RR_end: Interval Test RRy/uplimit
      mask DialogControl text_whl Prompt: Wheel
      mask DialogControl text_FL Prompt: FL
      mask DialogControl text_FR Prompt: FR
      mask DialogControl text_RL Prompt: RL
      mask DialogControl text_RR Prompt: RR
      mask DialogControl text_mu Prompt: Scale outside patch
      mask DialogControl text_mu_intv Prompt: Scale inside patch
      mask DialogControl text_x_start Prompt: Patch min X (m)
      mask DialogControl text_x_end Prompt: Patch max X (m)
      mask DialogControl text_y_start Prompt: Patch min Y (m)
      mask DialogControl text_y_end Prompt: Patch max Y (m)
  Road Surface Height : Subsystem  Variant=on  VariantControlMode=label  LabelModeActiveChoice=None  mask(Road Surface Profile Signal Inputs (Two Axle)){}
      mask help:
      | Provides signals to apply motion or forces to tire.  Used for KnC tests, multi-post testrigs, and road height adjustments.
      |
      | Set active variant using Variant Label.
      settings: AttributesFormatString=%<LabelModeActiveChoice>
      mask Display: disp(' ')
  RdBus : Outport  VectorParamsAs1DForOutWhenUnconnected=off
  wires:
  VehBus/1 -> Bus Selector1/1
  Mu Scaling by Position/1(L1) -> Ground/6(TyreScaling FL)
  Bus Selector1/1 -> Road Surface Height/1(Chassis), Mu Scaling by Position/1(Chassis)  "<Chassis>"
  Mu Scaling by Position/4(R2) -> Ground/9(TyreScaling RR)
  Road Surface Height/1(gz) -> Ground/1(gz)
  Mu Scaling by Position/3(L2) -> Ground/8(TyreScaling RL)
  Bus Creator/1 -> RdBus/1
  Mu Scaling by Position/2(R1) -> Ground/7(TyreScaling FR)
  Ground/1(L1) -> Bus Creator/1
  Ground/2(R1) -> Bus Creator/2
  Ground/3(L2) -> Bus Creator/3
  Ground/4(R2) -> Bus Creator/4
  Input fWindCar/1(fWind) -> Bus Creator/5  "fWindCar"
  Input fWindTrailer/1(fWind) -> Bus Creator/6  "fWindTrailer"
  Road Surface Height/2(uvec) -> Ground/2(uvec)
  Road Surface Height/3(fcp) -> Ground/3(fcp)
  Road Surface Height/4(fco) -> Ground/4(fco)
  Road Surface Height/5(fwc) -> Ground/5(fwc)

== system sm_car/Scopes ==
  Bus : Inport
  Bus Selector : BusSelector  OutputSignals=Chassis.WhlL1.aSlip,Chassis.WhlR1.aSlip,Chassis.WhlL2.aSlip,Chassis.WhlR2.aSlip
  Bus Selector1 : BusSelector  OutputSignals=Chassis.Spring.L1.xSpring,Chassis.Spring.R1.xSpring,Chassis.Spring.L2.xSpring,Chassis.Spring.R2.xSpring
  Bus Selector2 : BusSelector  OutputSignals=Chassis.WhlL1.Fx,Chassis.WhlR1.Fx,Chassis.WhlL2.Fx,Chassis.WhlR2.Fx
  Bus Selector3 : BusSelector  OutputSignals=Chassis.WhlL1.qxyz
  Bus Selector4 : BusSelector  OutputSignals=Driveline.anDriveshaftL1.q,Driveline.anDriveshaftR1.q,Driveline.anDriveshaftL1.w,Driveline.anDriveshaftR1.w
  Bus Selector5 : BusSelector  OutputSignals=Chassis.Body.CG.aRoll,Chassis.Body.CG.nRoll,Chassis.Body.CG.aPitch,Chassis.Body.CG.nPitch
  Bus Selector6 : BusSelector  OutputSignals=Chassis.WhlL1.n,Chassis.WhlR1.n,Chassis.WhlR2.n,Chassis.WhlL2.n
  Bus Selector7 : BusSelector  OutputSignals=Chassis.Body.CG.z,World.z
  Mux : Mux  Inputs=2
  Scope{,1..2,5..6,8} (6 alike) : Scope  NumInputPorts=4
      Scope settings: ActiveDisplayYMinimum=-1.96294  ActiveDisplayYMaximum=1.96118
      Scope1 settings: ActiveDisplayYMinimum=0.59933  ActiveDisplayYMaximum=0.77014
      Scope2 settings: ActiveDisplayYMinimum=-8724.32507  ActiveDisplayYMaximum=8948.55481
      Scope5 settings: ActiveDisplayYMinimum=-1.84919  ActiveDisplayYMaximum=0.7981
      Scope6 settings: ActiveDisplayYMinimum=-6.1E-5  ActiveDisplayYMaximum=7E-6
      Scope8 settings: TimeSpan=3  ActiveDisplayYMinimum=-3.30213  ActiveDisplayYMaximum=31.49608  DataLoggingVariableName=ScopeData2
  Scope3 : Scope
      settings: ActiveDisplayYMinimum=-86.18516  ActiveDisplayYMaximum=775.52925
  Scope4 : Scope  NumInputPorts=2
      settings: ActiveDisplayYMinimum=5.81523  ActiveDisplayYMaximum=6.20079
  Scope7 : Scope  NumInputPorts=2
      settings: ActiveDisplayYMinimum=-5E-7  ActiveDisplayYMaximum=4.9E-6  DataLoggingVariableName=ScopeData2
  Scope9 : Scope  NumInputPorts=2
      settings: ActiveDisplayYMinimum=-1.17425  ActiveDisplayYMaximum=10.16971
  Subsystem : Subsystem
  Transfer Fcn : TransferFcn  Numerator=[1 0]  Denominator=[0.01 1]
  xvCar : Outport  VectorParamsAs1DForOutWhenUnconnected=off
  wires:
  Bus/1 -> Bus Selector1/1, Bus Selector2/1, Bus Selector5/1, Bus Selector/1, Bus Selector7/1, Subsystem/1(In1), Bus Selector6/1, Bus Selector4/1, Bus Selector3/1
  Bus Selector/1 -> Scope/1  "<aSlip>"
  Bus Selector/2 -> Scope/2  "<aSlip>"
  Bus Selector/3 -> Scope/3  "<aSlip>"
  Bus Selector/4 -> Scope/4  "<aSlip>"
  Bus Selector1/1 -> Scope1/1  "<xSpring>"
  Bus Selector1/2 -> Scope1/2  "<xSpring>"
  Bus Selector1/3 -> Scope1/3  "<xSpring>"
  Bus Selector1/4 -> Scope1/4  "<xSpring>"
  Bus Selector2/3 -> Scope2/3  "<Fx>"
  Bus Selector2/4 -> Scope2/4  "<Fx>"
  Bus Selector2/2 -> Scope2/2  "<Fx>"
  Bus Selector2/1 -> Scope2/1  "<Fx>"
  Bus Selector3/1 -> Scope3/1  "<qxyz>"
  Subsystem/1(vBody) -> Scope4/1  "Body"
  Subsystem/2(vWorld) -> Mux/1, Scope4/2  "World"
  Mux/1 -> xvCar/1
  Subsystem/3(xWorld) -> Mux/2
  Bus Selector4/2 -> Scope5/2  "<q>"
  Bus Selector4/1 -> Scope5/1  "<q>"
  Bus Selector4/3 -> Scope5/3  "<w>"
  Bus Selector4/4 -> Scope5/4  "<w>"
  Bus Selector5/1 -> Scope6/1, Transfer Fcn/1  "<aRoll>"
  Bus Selector5/2 -> Scope7/2, Scope6/2  "<nRoll>"
  Bus Selector5/3 -> Scope6/3  "<aPitch>"
  Bus Selector5/4 -> Scope6/4  "<nPitch>"
  Transfer Fcn/1 -> Scope7/1
  Bus Selector6/1 -> Scope8/1  "<n>"
  Bus Selector6/2 -> Scope8/2  "<n>"
  Bus Selector6/3 -> Scope8/3  "<n>"
  Bus Selector6/4 -> Scope8/4  "<n>"
  Bus Selector7/1 -> Scope9/1  "<z>"
  Bus Selector7/2 -> Scope9/2  "<z>"

== system sm_car/Vehicle ==
  RdBus : Inport
  DrvBus : Inport  Port=2
  CtrlBus : Inport  Port=3
  CtrlBus1 : InportShadow  Port=3
  DrvBus1 : InportShadow  Port=2
  RdBus1 : InportShadow
  Trailer : Subsystem  Variant=on  VariantControlMode=label  VariantControl=NS_Con  LabelModeActiveChoice=None  mask(Variants for Trailer){veh_index=61}
      mask prompts: veh_index "Vehicle Index (for tires)"
      mask help: Enable or disable trailer. Set tire index to ensures tire results can be saved independently from other vehicles in the model. Change value of Initialization Trigger Dropdown to trigger selection of variant subsystems at this level and below.
      settings: AttributesFormatString=%<LabelModeActiveChoice>
      mask TypeOptions veh_index: Trailer/veh_index
      mask Display:
      | % Determine mask image to be displayed if Trailer is active
      | if(strcmpi(get_param(gcb,'LabelModeActiveChoice'),'Trailer'))
      | 
      |     % Get image from BodyGeometry.class
      |     % (active choice for Body Geometry subsystem)
      |     temp_veh_bg_class = lower(get_param([gcb '/Trailer/Chassis/Body/Body Geometry'],'LabelModeActiveChoice'));
      | 
      |     imagestr = (['sm_car_vehicle_' temp_veh_bg_class '.png']);
      |     if(~exist(imagestr))
      |         imagestr = ['sm_car_vehicle_axle1_default.png'];
      |     end
      | 
      |     image(imagestr);
      | 
      | end
  Vehicle : Subsystem  Tag=PublishSubsystem  VariantControl=NS_Con  mask(Vehicle with Two Axles){popup_BodyToWorld=Free, popup_wheel_spin=Free, Vehicle=Vehicle, Init=Init, SpecifyPosTarget=on, veh_index=1, mask_image_name=sm_car_vehicle_hamba_IMAGE.png}
      mask prompts: popup_BodyToWorld "Body To World Connection"; popup_wheel_spin "Wheel Spin"; Vehicle "Vehicle Parameters"; Init "Initial Values"; SpecifyPosTarget "Specify Position Target"; veh_index "Vehicle Index (for tires)"; mask_image_name "Mask Image (string)"
      mask help: Vehicle model with multibody suspension. Initial Values data structure sets initial speed of vehicle and wheels. Set tire index to ensure tire results can be saved independently from other vehicles in the model.
      mask Help: web('sm_car_doc_vehicle.html')
      mask TypeOptions popup_BodyToWorld: Body to World/popup_BodyToWorld
      mask TypeOptions popup_wheel_spin: Wheel Spin/popup_wheel_spin
      mask TypeOptions SpecifyPosTarget: Body to World/SpecifyPosTarget
      mask TypeOptions veh_index: Chassis/veh_index
      mask DialogControl cont_sim Prompt: Config
      mask DialogControl cont_connections Prompt: Lock for KnC Test
      mask Display:
      | % Get image from BodyGeometry.class
      | % (active choice for Body Geometry subsystem)
      | temp_veh_bg_class = lower(get_param([gcb '/Chassis/Body/Body Geometry'],'LabelModeActiveChoice'));
      | 
      | imagestr = (['sm_car_vehicle_' temp_veh_bg_class '.png']);
      | if(~exist(imagestr))
      |     imagestr = ['sm_car_vehicle_axle2_default.png'];
      | end
      | 
      | image(imagestr);
  Vehicle Constraint : Subsystem  Variant=on  VariantControlMode=label  VariantControl=Choice  LabelModeActiveChoice=NoConstraint
      settings: AttributesFormatString=%<LabelModeActiveChoice>
      mask Display: disp(' ');
  World Frame : sm_lib/Frames and Transforms/World Frame
  C : PMIOPort  Side=Left
  W : PMIOPort  Port=2  Side=Left
  TrlBus : Outport  VectorParamsAs1DForOutWhenUnconnected=off
  VehBus : Outport  Port=2  VectorParamsAs1DForOutWhenUnconnected=off
  wires:
  DrvBus/1 -> Vehicle/2(DrvBus)
  CtrlBus/1 -> Vehicle/3(CtrlBus)
  Vehicle/1(VehBus) -> VehBus/1
  RdBus/1 -> Vehicle/1(RdBus)
  RdBus1/1 -> Trailer/1("RdBus ")
  DrvBus1/1 -> Trailer/2("DrvBus ")
  CtrlBus1/1 -> Trailer/3("CtrlBus ")
  Trailer/1(" VehBus") -> TrlBus/1
  connections:
  Vehicle/LConn1 -- C/RConn1
  W/RConn1 -- Vehicle/LConn2
  Trailer/LConn2 -- Vehicle Constraint/LConn1 -- World Frame/RConn1
  Trailer/RConn1 -- Vehicle Constraint/RConn1 -- Vehicle/LConn3

== system sm_car/Visualization ==
  DrvBus : Inport
  VehBus : Inport  Port=2
  Bus Creator : BusCreator  Inputs=5
  Dashboard : Subsystem
  Data for Unreal : Subsystem
  Terminator : Terminator
  Unreal : Subsystem  Variant=on  VariantControlMode=label  VariantControl=Variant1  LabelModeActiveChoice=Off  mask{popup_animation=Off}
      mask prompts: popup_animation "Animation"
      mask init:
      | set_param(gcb,'LabelModeActiveChoice',get_param(gcb,'popup_animation'));
      settings: AttributesFormatString=%<LabelModeActiveChoice>
      mask TypeOptions popup_animation: Off | On
      mask Display: disp(' ');
  wires:
  DrvBus/1 -> Data for Unreal/2(DrvBus), Dashboard/2(DrvBus)
  VehBus/1 -> Data for Unreal/1(VehBus), Dashboard/1(VehBus)
  Data for Unreal/1(xyz) -> Bus Creator/1, Unreal/1("xyz ")  "xyz"
  Data for Unreal/2(rpy) -> Bus Creator/2, Unreal/2("rpy ")  "rpy"
  Data for Unreal/3(ws) -> Bus Creator/3, Unreal/3("ws ")  "ws"
  Data for Unreal/4(aCamber) -> Bus Creator/4, Unreal/4("aCamber ")  "aCamber"
  Data for Unreal/5(aSteerWheel) -> Bus Creator/5, Unreal/5("aSteerWheel ")  "aSteerWheel"
  Bus Creator/1 -> Terminator/1  "Unreal_Timeseries"

== system sm_car/World ==
  Mechanism Configuration : Subsystem  Variant=on  VariantControlMode=label  VariantControl=Choice  LabelModeActiveChoice=ConstantGravity
      settings: AttributesFormatString=%<LabelModeActiveChoice>
      mask Display: disp(' ');
  Scene : Subsystem  Variant=on  VariantControlMode=label  LabelModeActiveChoice=CRG_Hockenheim_F
      settings: AttributesFormatString=%<LabelModeActiveChoice>
  Solver Configuration : nesl_utility/Solver Configuration  PhysicalDomain=network_engine_domain  SubClassName=solver  LeftPortType=input  RightPortType=generic  Tones=[]  Harmonics=[]  SimulateNoise=off  Profile=off  UseLocalSampling=off  EnableSwitchedLinearOptims=on  FrequencyDomain=off  UseCCode=off  RelTol=0.001  AbsTol=1e-06  MinStep=1e-09  ToWorkspace=off  RevertToSquareIcSolve=off  NumHomotopyIterations=100  PhasorMode=off  PhasorModeNumHarmonics=1  ConsistencySolver=NEWTON_FTOL  IndexReductionMethod=DerivativeReplacement  DoDC=off  ResidualTolerance=1e-9  ConsistencyTolSource=GLOBAL  ConsistencyAbsTol=0.001  ConsistencyRelTol=0.001  ConsistencyTolFactor=0.001  UseLocalSolver=off  LocalSolverChoice=NE_BACKWARD_EULER_ADVANCER  ResolveIndetEquations=on  FunctionEvalNumThread=1  LocalSolverSampleTime=LocalSolverSampleTime  DoFixedCost=off  MaxNonlinIter=MaxNonlinIter  MaxModeIter=2  ComputeImpulses=off  ImpulseIterations=2  LinearAlgebra=Sparse  LinearAlgebraNumThread=0  EquationFormulation=NE_TIME_EF  DelaysMemoryBudget=1024  AutomaticFiltering=on  FilteringTimeConstant=0.001  PartitionStorageMethod=AS_NEEDED  PartitionMemoryBudget=1024  PartitionMethod=FAST  MultibodyUseLocalSolver=off  MultibodyLocalSolverChoice=ODE1  MultibodyLocalSolverSampleTime=0.001
  Visuals : Subsystem  Variant=on  VariantControlMode=label  VariantControl=Choice  LabelModeActiveChoice=Off  mask{popup_vis_point=Off, time_vector=time_vector, xyz_matrix=xyz_matrix, clr_vis=clr_vis, opc_vis=opc_vis, rad_vis=rad_vis}
      mask prompts: popup_vis_point "Visualize Point"; time_vector "Time Vector [nx1] (sec)"; xyz_matrix "Coordinates [nx3] (m)"; clr_vis "Color [R G B] (0-1)"; opc_vis "Opacity (0-1)"; rad_vis "Radius (m)"
      mask init:
      | bh = gcb;
      | pvisPt = get_param(bh,'popup_vis_point');
      | if(strcmp(pvisPt,'Off'))
      |     time_vector = [0];
      |     xyz_matrix =  [0 0 0];
      | end
      | set_param(bh,'LabelModeActiveChoice',pvisPt)
      mask TypeOptions popup_vis_point: Off | On
      mask Callback popup_vis_point:
      | bh = gcb;
      | maskObj = Simulink.Mask.get(bh); % Get the mask object of the current block
      | tvec_h  = maskObj.getParameter('time_vector'); % Get the parameter to hide
      | xyz_h   = maskObj.getParameter('xyz_matrix'); % Get the parameter to hide
      | clr_h   = maskObj.getParameter('clr_vis'); % Get the parameter to hide
      | opc_h   = maskObj.getParameter('opc_vis'); % Get the parameter to hide
      | rad_h   = maskObj.getParameter('rad_vis'); % Get the parameter to hide
      | 
      | % Check the value of ControlParam
      | enaVisPnt = get_param(bh, 'popup_vis_point');
      | 
      | tvec_h.Visible  = 'off';
      | xyz_h.Visible  = 'off';
      | clr_h.Visible  = 'off';
      | opc_h.Visible  = 'off';
      | rad_h.Visible  = 'off';
      | 
      | if strcmp(enaVisPnt, 'On')
      |     tvec_h.Visible  = 'on';
      |     xyz_h.Visible   = 'on';
      |     clr_h.Visible   = 'on';
      |     opc_h.Visible   = 'on';
      |     rad_h.Visible   = 'on';
      | end
  World Frame : sm_lib/Frames and Transforms/World Frame
  W : PMIOPort  Side=Left
  Obs : Outport  VectorParamsAs1DForOutWhenUnconnected=off
  wires:
  Scene/1(Obs) -> Obs/1
  connections:
  Scene/LConn1 -- W/RConn1 -- World Frame/RConn1 -- Visuals/LConn1 -- Mechanism Configuration/RConn1 -- Solver Configuration/RConn1

== system sm_car/Camera Frames/Dolly Camera ==
  Off : Subsystem  VariantControl=Off  mask{tvec=Camera.Dolly_Cam.tvec.Value, xvec=Camera.Dolly_Cam.xvec.Value, yvec=Camera.Dolly_Cam.yvec.Value, zvec=Camera.Dolly_Cam.zvec.Value, s=Camera.Dolly_Cam.s.Value, a=Camera.Dolly_Cam.a.Value}
      mask prompts: tvec "Time Vector (s)"; xvec "X Vector (m)"; yvec "Y Vector (m)"; zvec "Z Vector (m)"; s "Camera Offset [xyz] (m)"; a "Camera Orientation [Roll-Pitch-Yaw] (deg)"
  " W" : PMIOPort  Side=Left
  " R" : PMIOPort  Port=2  Side=Right

== system sm_car/Camera Frames/Transform FL ==
  Transform Camera Frame : sm_lib/Frames and Transforms/Rigid Transform  RotationMethod=RotationSequence  FollAlignAxisA=+X  BaseAlignAxisA=+Y  FollAlignAxisB=+Y  BaseAlignAxisB=+Z  RotationStandardAxis=+Z  RotationAngle=0.0  RotationAngleUnits=deg  RotationArbitraryAxis=[0 0 1]  RotationSequenceAxes=FollowerAxes  RotationSequence=ZYX  RotationSequenceAngles=CF.a.Value(3:-1:1)  RotationSequenceAnglesUnits=deg  RotationMatrix=[1 0 0; 0 1 0; 0 0 1]  Quaternion=[1 0 0 0]  TranslationMethod=Cartesian  TranslationCartesianOffset=CF.s.Value  TranslationCartesianOffsetUnits=m  TranslationStandardAxis=+Z  TranslationStandardOffset=0  TranslationStandardOffsetUnits=m  TranslationROffset=0  TranslationROffsetUnits=m  TranslationThetaOffset=0  TranslationThetaOffsetUnits=deg  TranslationZOffset=0  TranslationZOffsetUnits=m
  B : PMIOPort  Side=Left
  F : PMIOPort  Port=2  Side=Right
  connections:
  Transform Camera Frame/RConn1 -- F/RConn1
  Transform Camera Frame/LConn1 -- B/RConn1
